simulink model "skarab_fgbe"  (R2018a)
settings: Solver=VariableStepDiscrete  StartTime=0.0  StopTime=50000  RelTol=1e-3
libraries: xbsIndex_r4 x178, xps_library x3, casper_library_misc x2
(part 3 of 3)

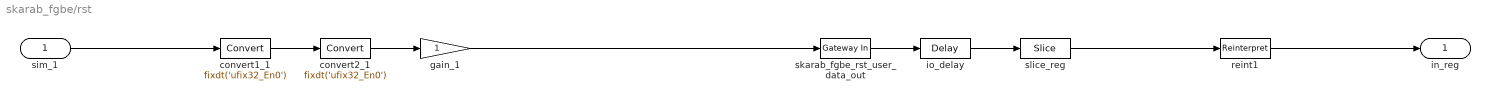
== system skarab_fgbe/rst ==
  sim_1 : Inport
  convert1_1 : DataTypeConversion  OutDataTypeStr=fixdt('ufix32_En0')  LockScale=on
  convert2_1 : DataTypeConversion  OutDataTypeStr=fixdt('ufix32_En0')  ConvertRealWorld=Stored Integer (SI)  LockScale=on
  gain_1 : Gain
  io_delay : xbsIndex_r4/Delay  rst=off  infoeditControl=Selection of Reset will increase slice count due to use of real FFs and instead of SRLs  en=off  latency=0  reg_retiming=on  dbl_ovrd=off  block_type=delay
  reint1 : xbsIndex_r4/Reinterpret  force_arith_type=on  arith_type=Unsigned  force_bin_pt=on  bin_pt=0  block_type=reinterpret
  skarab_fgbe_rst_user_data_out : xbsIndex_r4/Gateway In  gui_display_data_type=Fixed-point  arith_type=Unsigned  n_bits=32  bin_pt=0  preci_type=Single  exp_width=8  frac_width=24  rows=1  columns=1  quantization="Round  (unbiased: +/- Inf)"  overflow=Saturate  period=1  UseAsADC=off  ADCChannel='1'  interface=None  automatic_assignment=on  address_offset=hex2dec('00')  intf_name=''  intf_description=''  default_value=0  timing_constraint=None  locs_specified=off  LOCs={}  io_standard={}  inherit_from_input=off  hdl_port=on  dbl_ovrd=off  block_type=gatewayin
  slice_reg : xbsIndex_r4/Slice  nbits=32  boolean_output=off  mode=Lower Bit Location + Width  bit1=0  base1=MSB of Input  bit0=0  base0=LSB of Input  dbl_ovrd=off  block_type=slice
  in_reg : Outport
  wires:
  skarab_fgbe_rst_user_data_out/1 -> io_delay/1
  sim_1/1 -> convert1_1/1
  convert1_1/1 -> convert2_1/1
  convert2_1/1 -> gain_1/1
  gain_1/1 -> skarab_fgbe_rst_user_data_out/1
  io_delay/1 -> slice_reg/1
  slice_reg/1 -> reint1/1
  reint1/1 -> in_reg/1

== system skarab_fgbe/rx ==
  out_reg : Inport
  assert_reg : xbsIndex_r4/Assert  assert_type=on  type_source=Explicitly  gui_display_data_type=Fixed-point  arith_type=Unsigned  n_bits=32  bin_pt=0  preci_type=Single  exp_width=8  frac_width=24  assert_rate=off  rate_source=Explicitly  period=1  output_port=on  block_type=assert
  cast_gw : xbsIndex_r4/Convert  gui_display_data_type=Fixed-point  arith_type=Unsigned  n_bits=32  bin_pt=0  float_type=Single  exp_bits=8  fraction_bits=24  quantization=Truncate  overflow=Wrap  en=off  latency=1  pipeline=off  dbl_ovrd=off  block_type=convert
  io_delay : xbsIndex_r4/Delay  rst=off  infoeditControl=Selection of Reset will increase slice count due to use of real FFs and instead of SRLs  en=off  latency=0  reg_retiming=on  dbl_ovrd=off  block_type=delay
  reint1 : xbsIndex_r4/Reinterpret  force_arith_type=on  arith_type=Unsigned  force_bin_pt=on  bin_pt=0  block_type=reinterpret
  skarab_fgbe_rx_user_data_in : xbsIndex_r4/Gateway Out  inherit_from_input=off  hdl_port=on  rows=1  columns=1  UseAsDAC=off  DACChannel='1'  interface=None  automatic_assignment=on  address_offset=hex2dec('00')  intf_name=''  intf_description=''  timing_constraint=None  locs_specified=off  LOCs={}  io_standard={}  block_type=gatewayout
  sim_out : Outport
  wires:
  io_delay/1 -> cast_gw/1
  cast_gw/1 -> skarab_fgbe_rx_user_data_in/1
  skarab_fgbe_rx_user_data_in/1 -> sim_out/1
  out_reg/1 -> assert_reg/1
  assert_reg/1 -> reint1/1
  reint1/1 -> io_delay/1

== system skarab_fgbe/rx_bad_frame ==
  out_reg : Inport
  assert_reg : xbsIndex_r4/Assert  assert_type=on  type_source=Explicitly  gui_display_data_type=Fixed-point  arith_type=Unsigned  n_bits=32  bin_pt=0  preci_type=Single  exp_width=8  frac_width=24  assert_rate=off  rate_source=Explicitly  period=1  output_port=on  block_type=assert
  cast_gw : xbsIndex_r4/Convert  gui_display_data_type=Fixed-point  arith_type=Unsigned  n_bits=32  bin_pt=0  float_type=Single  exp_bits=8  fraction_bits=24  quantization=Truncate  overflow=Wrap  en=off  latency=1  pipeline=off  dbl_ovrd=off  block_type=convert
  io_delay : xbsIndex_r4/Delay  rst=off  infoeditControl=Selection of Reset will increase slice count due to use of real FFs and instead of SRLs  en=off  latency=0  reg_retiming=on  dbl_ovrd=off  block_type=delay
  reint1 : xbsIndex_r4/Reinterpret  force_arith_type=on  arith_type=Unsigned  force_bin_pt=on  bin_pt=0  block_type=reinterpret
  skarab_fgbe_rx_bad_frame_user_data_in : xbsIndex_r4/Gateway Out  inherit_from_input=off  hdl_port=on  rows=1  columns=1  UseAsDAC=off  DACChannel='1'  interface=None  automatic_assignment=on  address_offset=hex2dec('00')  intf_name=''  intf_description=''  timing_constraint=None  locs_specified=off  LOCs={}  io_standard={}  block_type=gatewayout
  sim_out : Outport
  wires:
  io_delay/1 -> cast_gw/1
  cast_gw/1 -> skarab_fgbe_rx_bad_frame_user_data_in/1
  skarab_fgbe_rx_bad_frame_user_data_in/1 -> sim_out/1
  out_reg/1 -> assert_reg/1
  assert_reg/1 -> reint1/1
  reint1/1 -> io_delay/1

== system skarab_fgbe/rx_data ==
  out_reg : Inport
  assert_reg : xbsIndex_r4/Assert  assert_type=on  type_source=Explicitly  gui_display_data_type=Fixed-point  arith_type=Unsigned  n_bits=32  bin_pt=0  preci_type=Single  exp_width=8  frac_width=24  assert_rate=off  rate_source=Explicitly  period=1  output_port=on  block_type=assert
  cast_gw : xbsIndex_r4/Convert  gui_display_data_type=Fixed-point  arith_type=Unsigned  n_bits=32  bin_pt=0  float_type=Single  exp_bits=8  fraction_bits=24  quantization=Truncate  overflow=Wrap  en=off  latency=1  pipeline=off  dbl_ovrd=off  block_type=convert
  io_delay : xbsIndex_r4/Delay  rst=off  infoeditControl=Selection of Reset will increase slice count due to use of real FFs and instead of SRLs  en=off  latency=0  reg_retiming=on  dbl_ovrd=off  block_type=delay
  reint1 : xbsIndex_r4/Reinterpret  force_arith_type=on  arith_type=Unsigned  force_bin_pt=on  bin_pt=0  block_type=reinterpret
  skarab_fgbe_rx_data_user_data_in : xbsIndex_r4/Gateway Out  inherit_from_input=off  hdl_port=on  rows=1  columns=1  UseAsDAC=off  DACChannel='1'  interface=None  automatic_assignment=on  address_offset=hex2dec('00')  intf_name=''  intf_description=''  timing_constraint=None  locs_specified=off  LOCs={}  io_standard={}  block_type=gatewayout
  sim_out : Outport
  wires:
  io_delay/1 -> cast_gw/1
  cast_gw/1 -> skarab_fgbe_rx_data_user_data_in/1
  skarab_fgbe_rx_data_user_data_in/1 -> sim_out/1
  out_reg/1 -> assert_reg/1
  assert_reg/1 -> reint1/1
  reint1/1 -> io_delay/1

== system skarab_fgbe/rx_dest_ip ==
  out_reg : Inport
  assert_reg : xbsIndex_r4/Assert  assert_type=on  type_source=Explicitly  gui_display_data_type=Fixed-point  arith_type=Unsigned  n_bits=32  bin_pt=0  preci_type=Single  exp_width=8  frac_width=24  assert_rate=off  rate_source=Explicitly  period=1  output_port=on  block_type=assert
  cast_gw : xbsIndex_r4/Convert  gui_display_data_type=Fixed-point  arith_type=Unsigned  n_bits=32  bin_pt=0  float_type=Single  exp_bits=8  fraction_bits=24  quantization=Truncate  overflow=Wrap  en=off  latency=1  pipeline=off  dbl_ovrd=off  block_type=convert
  io_delay : xbsIndex_r4/Delay  rst=off  infoeditControl=Selection of Reset will increase slice count due to use of real FFs and instead of SRLs  en=off  latency=0  reg_retiming=on  dbl_ovrd=off  block_type=delay
  reint1 : xbsIndex_r4/Reinterpret  force_arith_type=on  arith_type=Unsigned  force_bin_pt=on  bin_pt=0  block_type=reinterpret
  skarab_fgbe_rx_dest_ip_user_data_in : xbsIndex_r4/Gateway Out  inherit_from_input=off  hdl_port=on  rows=1  columns=1  UseAsDAC=off  DACChannel='1'  interface=None  automatic_assignment=on  address_offset=hex2dec('00')  intf_name=''  intf_description=''  timing_constraint=None  locs_specified=off  LOCs={}  io_standard={}  block_type=gatewayout
  sim_out : Outport
  wires:
  io_delay/1 -> cast_gw/1
  cast_gw/1 -> skarab_fgbe_rx_dest_ip_user_data_in/1
  skarab_fgbe_rx_dest_ip_user_data_in/1 -> sim_out/1
  out_reg/1 -> assert_reg/1
  assert_reg/1 -> reint1/1
  reint1/1 -> io_delay/1

== system skarab_fgbe/rx_dest_port ==
  out_reg : Inport
  assert_reg : xbsIndex_r4/Assert  assert_type=on  type_source=Explicitly  gui_display_data_type=Fixed-point  arith_type=Unsigned  n_bits=32  bin_pt=0  preci_type=Single  exp_width=8  frac_width=24  assert_rate=off  rate_source=Explicitly  period=1  output_port=on  block_type=assert
  cast_gw : xbsIndex_r4/Convert  gui_display_data_type=Fixed-point  arith_type=Unsigned  n_bits=32  bin_pt=0  float_type=Single  exp_bits=8  fraction_bits=24  quantization=Truncate  overflow=Wrap  en=off  latency=1  pipeline=off  dbl_ovrd=off  block_type=convert
  io_delay : xbsIndex_r4/Delay  rst=off  infoeditControl=Selection of Reset will increase slice count due to use of real FFs and instead of SRLs  en=off  latency=0  reg_retiming=on  dbl_ovrd=off  block_type=delay
  reint1 : xbsIndex_r4/Reinterpret  force_arith_type=on  arith_type=Unsigned  force_bin_pt=on  bin_pt=0  block_type=reinterpret
  skarab_fgbe_rx_dest_port_user_data_in : xbsIndex_r4/Gateway Out  inherit_from_input=off  hdl_port=on  rows=1  columns=1  UseAsDAC=off  DACChannel='1'  interface=None  automatic_assignment=on  address_offset=hex2dec('00')  intf_name=''  intf_description=''  timing_constraint=None  locs_specified=off  LOCs={}  io_standard={}  block_type=gatewayout
  sim_out : Outport
  wires:
  io_delay/1 -> cast_gw/1
  cast_gw/1 -> skarab_fgbe_rx_dest_port_user_data_in/1
  skarab_fgbe_rx_dest_port_user_data_in/1 -> sim_out/1
  out_reg/1 -> assert_reg/1
  assert_reg/1 -> reint1/1
  reint1/1 -> io_delay/1

== system skarab_fgbe/rx_end_of_frame ==
  out_reg : Inport
  assert_reg : xbsIndex_r4/Assert  assert_type=on  type_source=Explicitly  gui_display_data_type=Fixed-point  arith_type=Unsigned  n_bits=32  bin_pt=0  preci_type=Single  exp_width=8  frac_width=24  assert_rate=off  rate_source=Explicitly  period=1  output_port=on  block_type=assert
  cast_gw : xbsIndex_r4/Convert  gui_display_data_type=Fixed-point  arith_type=Unsigned  n_bits=32  bin_pt=0  float_type=Single  exp_bits=8  fraction_bits=24  quantization=Truncate  overflow=Wrap  en=off  latency=1  pipeline=off  dbl_ovrd=off  block_type=convert
  io_delay : xbsIndex_r4/Delay  rst=off  infoeditControl=Selection of Reset will increase slice count due to use of real FFs and instead of SRLs  en=off  latency=0  reg_retiming=on  dbl_ovrd=off  block_type=delay
  reint1 : xbsIndex_r4/Reinterpret  force_arith_type=on  arith_type=Unsigned  force_bin_pt=on  bin_pt=0  block_type=reinterpret
  skarab_fgbe_rx_end_of_frame_user_data_in : xbsIndex_r4/Gateway Out  inherit_from_input=off  hdl_port=on  rows=1  columns=1  UseAsDAC=off  DACChannel='1'  interface=None  automatic_assignment=on  address_offset=hex2dec('00')  intf_name=''  intf_description=''  timing_constraint=None  locs_specified=off  LOCs={}  io_standard={}  block_type=gatewayout
  sim_out : Outport
  wires:
  io_delay/1 -> cast_gw/1
  cast_gw/1 -> skarab_fgbe_rx_end_of_frame_user_data_in/1
  skarab_fgbe_rx_end_of_frame_user_data_in/1 -> sim_out/1
  out_reg/1 -> assert_reg/1
  assert_reg/1 -> reint1/1
  reint1/1 -> io_delay/1

== system skarab_fgbe/rx_valid ==
  out_reg : Inport
  assert_reg : xbsIndex_r4/Assert  assert_type=on  type_source=Explicitly  gui_display_data_type=Fixed-point  arith_type=Unsigned  n_bits=32  bin_pt=0  preci_type=Single  exp_width=8  frac_width=24  assert_rate=off  rate_source=Explicitly  period=1  output_port=on  block_type=assert
  cast_gw : xbsIndex_r4/Convert  gui_display_data_type=Fixed-point  arith_type=Unsigned  n_bits=32  bin_pt=0  float_type=Single  exp_bits=8  fraction_bits=24  quantization=Truncate  overflow=Wrap  en=off  latency=1  pipeline=off  dbl_ovrd=off  block_type=convert
  io_delay : xbsIndex_r4/Delay  rst=off  infoeditControl=Selection of Reset will increase slice count due to use of real FFs and instead of SRLs  en=off  latency=0  reg_retiming=on  dbl_ovrd=off  block_type=delay
  reint1 : xbsIndex_r4/Reinterpret  force_arith_type=on  arith_type=Unsigned  force_bin_pt=on  bin_pt=0  block_type=reinterpret
  skarab_fgbe_rx_valid_user_data_in : xbsIndex_r4/Gateway Out  inherit_from_input=off  hdl_port=on  rows=1  columns=1  UseAsDAC=off  DACChannel='1'  interface=None  automatic_assignment=on  address_offset=hex2dec('00')  intf_name=''  intf_description=''  timing_constraint=None  locs_specified=off  LOCs={}  io_standard={}  block_type=gatewayout
  sim_out : Outport
  wires:
  io_delay/1 -> cast_gw/1
  cast_gw/1 -> skarab_fgbe_rx_valid_user_data_in/1
  skarab_fgbe_rx_valid_user_data_in/1 -> sim_out/1
  out_reg/1 -> assert_reg/1
  assert_reg/1 -> reint1/1
  reint1/1 -> io_delay/1

== system skarab_fgbe/tx ==
  out_reg : Inport
  assert_reg : xbsIndex_r4/Assert  assert_type=on  type_source=Explicitly  gui_display_data_type=Fixed-point  arith_type=Unsigned  n_bits=32  bin_pt=0  preci_type=Single  exp_width=8  frac_width=24  assert_rate=off  rate_source=Explicitly  period=1  output_port=on  block_type=assert
  cast_gw : xbsIndex_r4/Convert  gui_display_data_type=Fixed-point  arith_type=Unsigned  n_bits=32  bin_pt=0  float_type=Single  exp_bits=8  fraction_bits=24  quantization=Truncate  overflow=Wrap  en=off  latency=1  pipeline=off  dbl_ovrd=off  block_type=convert
  io_delay : xbsIndex_r4/Delay  rst=off  infoeditControl=Selection of Reset will increase slice count due to use of real FFs and instead of SRLs  en=off  latency=0  reg_retiming=on  dbl_ovrd=off  block_type=delay
  reint1 : xbsIndex_r4/Reinterpret  force_arith_type=on  arith_type=Unsigned  force_bin_pt=on  bin_pt=0  block_type=reinterpret
  skarab_fgbe_tx_user_data_in : xbsIndex_r4/Gateway Out  inherit_from_input=off  hdl_port=on  rows=1  columns=1  UseAsDAC=off  DACChannel='1'  interface=None  automatic_assignment=on  address_offset=hex2dec('00')  intf_name=''  intf_description=''  timing_constraint=None  locs_specified=off  LOCs={}  io_standard={}  block_type=gatewayout
  sim_out : Outport
  wires:
  io_delay/1 -> cast_gw/1
  cast_gw/1 -> skarab_fgbe_tx_user_data_in/1
  skarab_fgbe_tx_user_data_in/1 -> sim_out/1
  out_reg/1 -> assert_reg/1
  assert_reg/1 -> reint1/1
  reint1/1 -> io_delay/1

== system skarab_fgbe/tx_cnt ==
  out_reg : Inport
  assert_reg : xbsIndex_r4/Assert  assert_type=on  type_source=Explicitly  gui_display_data_type=Fixed-point  arith_type=Unsigned  n_bits=32  bin_pt=0  preci_type=Single  exp_width=8  frac_width=24  assert_rate=off  rate_source=Explicitly  period=1  output_port=on  block_type=assert
  cast_gw : xbsIndex_r4/Convert  gui_display_data_type=Fixed-point  arith_type=Unsigned  n_bits=32  bin_pt=0  float_type=Single  exp_bits=8  fraction_bits=24  quantization=Truncate  overflow=Wrap  en=off  latency=1  pipeline=off  dbl_ovrd=off  block_type=convert
  io_delay : xbsIndex_r4/Delay  rst=off  infoeditControl=Selection of Reset will increase slice count due to use of real FFs and instead of SRLs  en=off  latency=0  reg_retiming=on  dbl_ovrd=off  block_type=delay
  reint1 : xbsIndex_r4/Reinterpret  force_arith_type=on  arith_type=Unsigned  force_bin_pt=on  bin_pt=0  block_type=reinterpret
  skarab_fgbe_tx_cnt_user_data_in : xbsIndex_r4/Gateway Out  inherit_from_input=off  hdl_port=on  rows=1  columns=1  UseAsDAC=off  DACChannel='1'  interface=None  automatic_assignment=on  address_offset=hex2dec('00')  intf_name=''  intf_description=''  timing_constraint=None  locs_specified=off  LOCs={}  io_standard={}  block_type=gatewayout
  sim_out : Outport
  wires:
  io_delay/1 -> cast_gw/1
  cast_gw/1 -> skarab_fgbe_tx_cnt_user_data_in/1
  skarab_fgbe_tx_cnt_user_data_in/1 -> sim_out/1
  out_reg/1 -> assert_reg/1
  assert_reg/1 -> reint1/1
  reint1/1 -> io_delay/1

== system skarab_fgbe/tx_full ==
  out_reg : Inport
  assert_reg : xbsIndex_r4/Assert  assert_type=on  type_source=Explicitly  gui_display_data_type=Fixed-point  arith_type=Unsigned  n_bits=32  bin_pt=0  preci_type=Single  exp_width=8  frac_width=24  assert_rate=off  rate_source=Explicitly  period=1  output_port=on  block_type=assert
  cast_gw : xbsIndex_r4/Convert  gui_display_data_type=Fixed-point  arith_type=Unsigned  n_bits=32  bin_pt=0  float_type=Single  exp_bits=8  fraction_bits=24  quantization=Truncate  overflow=Wrap  en=off  latency=1  pipeline=off  dbl_ovrd=off  block_type=convert
  io_delay : xbsIndex_r4/Delay  rst=off  infoeditControl=Selection of Reset will increase slice count due to use of real FFs and instead of SRLs  en=off  latency=0  reg_retiming=on  dbl_ovrd=off  block_type=delay
  reint1 : xbsIndex_r4/Reinterpret  force_arith_type=on  arith_type=Unsigned  force_bin_pt=on  bin_pt=0  block_type=reinterpret
  skarab_fgbe_tx_full_user_data_in : xbsIndex_r4/Gateway Out  inherit_from_input=off  hdl_port=on  rows=1  columns=1  UseAsDAC=off  DACChannel='1'  interface=None  automatic_assignment=on  address_offset=hex2dec('00')  intf_name=''  intf_description=''  timing_constraint=None  locs_specified=off  LOCs={}  io_standard={}  block_type=gatewayout
  sim_out : Outport
  wires:
  io_delay/1 -> cast_gw/1
  cast_gw/1 -> skarab_fgbe_tx_full_user_data_in/1
  skarab_fgbe_tx_full_user_data_in/1 -> sim_out/1
  out_reg/1 -> assert_reg/1
  assert_reg/1 -> reint1/1
  reint1/1 -> io_delay/1

== system skarab_fgbe/tx_overflow ==
  out_reg : Inport
  assert_reg : xbsIndex_r4/Assert  assert_type=on  type_source=Explicitly  gui_display_data_type=Fixed-point  arith_type=Unsigned  n_bits=32  bin_pt=0  preci_type=Single  exp_width=8  frac_width=24  assert_rate=off  rate_source=Explicitly  period=1  output_port=on  block_type=assert
  cast_gw : xbsIndex_r4/Convert  gui_display_data_type=Fixed-point  arith_type=Unsigned  n_bits=32  bin_pt=0  float_type=Single  exp_bits=8  fraction_bits=24  quantization=Truncate  overflow=Wrap  en=off  latency=1  pipeline=off  dbl_ovrd=off  block_type=convert
  io_delay : xbsIndex_r4/Delay  rst=off  infoeditControl=Selection of Reset will increase slice count due to use of real FFs and instead of SRLs  en=off  latency=0  reg_retiming=on  dbl_ovrd=off  block_type=delay
  reint1 : xbsIndex_r4/Reinterpret  force_arith_type=on  arith_type=Unsigned  force_bin_pt=on  bin_pt=0  block_type=reinterpret
  skarab_fgbe_tx_overflow_user_data_in : xbsIndex_r4/Gateway Out  inherit_from_input=off  hdl_port=on  rows=1  columns=1  UseAsDAC=off  DACChannel='1'  interface=None  automatic_assignment=on  address_offset=hex2dec('00')  intf_name=''  intf_description=''  timing_constraint=None  locs_specified=off  LOCs={}  io_standard={}  block_type=gatewayout
  sim_out : Outport
  wires:
  io_delay/1 -> cast_gw/1
  cast_gw/1 -> skarab_fgbe_tx_overflow_user_data_in/1
  skarab_fgbe_tx_overflow_user_data_in/1 -> sim_out/1
  out_reg/1 -> assert_reg/1
  assert_reg/1 -> reint1/1
  reint1/1 -> io_delay/1

== system skarab_fgbe/forty_gbe/convert_tx_valid ==
  in : Inport
  bussify : Subsystem  AncestorBlock=casper_library_flow_control/bus_create  mask(bus_create){inputNum=4}
      mask prompts: inputNum "Number of inputs:"
      mask init:
      | bus_create_init(gcb,...
      |     'inputNum', inputNum);
  out : Outport
  wires:
  in/1 -> bussify/1(in1), bussify/2(in2), bussify/3(in3), bussify/4(in4)
  bussify/1(bus_out) -> out/1

== system skarab_fgbe/forty_gbe/pipeline_led_rx ==
  d : Inport
  q : Outport
  wires:
  d/1 -> q/1

== system skarab_fgbe/forty_gbe/pipeline_led_tx ==
  d : Inport
  q : Outport
  wires:
  d/1 -> q/1

== system skarab_fgbe/forty_gbe/pipeline_led_up ==
  d : Inport
  q : Outport
  wires:
  d/1 -> q/1

== system skarab_fgbe/forty_gbe/pipeline_rx_bad_frame ==
  d : Inport
  q : Outport
  wires:
  d/1 -> q/1

== system skarab_fgbe/forty_gbe/pipeline_rx_data ==
  d : Inport
  q : Outport
  wires:
  d/1 -> q/1

== system skarab_fgbe/forty_gbe/pipeline_rx_dest_ip ==
  d : Inport
  q : Outport
  wires:
  d/1 -> q/1

== system skarab_fgbe/forty_gbe/pipeline_rx_dest_port ==
  d : Inport
  q : Outport
  wires:
  d/1 -> q/1

== system skarab_fgbe/forty_gbe/pipeline_rx_end_of_frame ==
  d : Inport
  q : Outport
  wires:
  d/1 -> q/1

== system skarab_fgbe/forty_gbe/pipeline_rx_overrun ==
  d : Inport
  q : Outport
  wires:
  d/1 -> q/1

== system skarab_fgbe/forty_gbe/pipeline_rx_source_ip ==
  d : Inport
  q : Outport
  wires:
  d/1 -> q/1

== system skarab_fgbe/forty_gbe/pipeline_rx_source_port ==
  d : Inport
  q : Outport
  wires:
  d/1 -> q/1

== system skarab_fgbe/forty_gbe/pipeline_rx_valid ==
  d : Inport
  q : Outport
  wires:
  d/1 -> q/1

== system skarab_fgbe/forty_gbe/pipeline_tx_afull ==
  d : Inport
  q : Outport
  wires:
  d/1 -> q/1

== system skarab_fgbe/forty_gbe/pipeline_tx_overflow ==
  d : Inport
  q : Outport
  wires:
  d/1 -> q/1

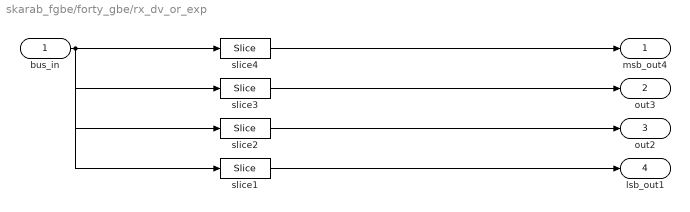
== system skarab_fgbe/forty_gbe/rx_dv_or_exp ==
  bus_in : Inport
  slice1 : xbsIndex_r4/Slice  nbits=1  boolean_output=on  mode=Upper Bit Location + Width  bit1=-3  base1=MSB of Input  bit0=0  base0=LSB of Input  dbl_ovrd=off  block_type=slice
  slice2 : xbsIndex_r4/Slice  nbits=1  boolean_output=on  mode=Upper Bit Location + Width  bit1=-2  base1=MSB of Input  bit0=0  base0=LSB of Input  dbl_ovrd=off  block_type=slice
  slice3 : xbsIndex_r4/Slice  nbits=1  boolean_output=on  mode=Upper Bit Location + Width  bit1=-1  base1=MSB of Input  bit0=0  base0=LSB of Input  dbl_ovrd=off  block_type=slice
  slice4 : xbsIndex_r4/Slice  nbits=1  boolean_output=on  mode=Upper Bit Location + Width  bit1=0  base1=MSB of Input  bit0=0  base0=LSB of Input  dbl_ovrd=off  block_type=slice
  msb_out4 : Outport
  out3 : Outport  Port=2
  out2 : Outport  Port=3
  lsb_out1 : Outport  Port=4
  wires:
  bus_in/1 -> slice4/1, slice3/1, slice2/1, slice1/1
  slice4/1 -> msb_out4/1
  slice3/1 -> out3/1
  slice2/1 -> out2/1
  slice1/1 -> lsb_out1/1

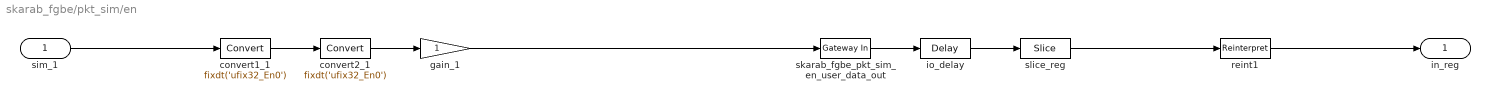
== system skarab_fgbe/pkt_sim/en ==
  sim_1 : Inport
  convert1_1 : DataTypeConversion  OutDataTypeStr=fixdt('ufix32_En0')  LockScale=on
  convert2_1 : DataTypeConversion  OutDataTypeStr=fixdt('ufix32_En0')  ConvertRealWorld=Stored Integer (SI)  LockScale=on
  gain_1 : Gain
  io_delay : xbsIndex_r4/Delay  rst=off  infoeditControl=Selection of Reset will increase slice count due to use of real FFs and instead of SRLs  en=off  latency=0  reg_retiming=on  dbl_ovrd=off  block_type=delay
  reint1 : xbsIndex_r4/Reinterpret  force_arith_type=on  arith_type=Unsigned  force_bin_pt=on  bin_pt=0  block_type=reinterpret
  skarab_fgbe_pkt_sim_en_user_data_out : xbsIndex_r4/Gateway In  gui_display_data_type=Fixed-point  arith_type=Unsigned  n_bits=32  bin_pt=0  preci_type=Single  exp_width=8  frac_width=24  rows=1  columns=1  quantization="Round  (unbiased: +/- Inf)"  overflow=Saturate  period=1  UseAsADC=off  ADCChannel='1'  interface=None  automatic_assignment=on  address_offset=hex2dec('00')  intf_name=''  intf_description=''  default_value=0  timing_constraint=None  locs_specified=off  LOCs={}  io_standard={}  inherit_from_input=off  hdl_port=on  dbl_ovrd=off  block_type=gatewayin
  slice_reg : xbsIndex_r4/Slice  nbits=32  boolean_output=off  mode=Lower Bit Location + Width  bit1=0  base1=MSB of Input  bit0=0  base0=LSB of Input  dbl_ovrd=off  block_type=slice
  in_reg : Outport
  wires:
  skarab_fgbe_pkt_sim_en_user_data_out/1 -> io_delay/1
  sim_1/1 -> convert1_1/1
  convert1_1/1 -> convert2_1/1
  convert2_1/1 -> gain_1/1
  gain_1/1 -> skarab_fgbe_pkt_sim_en_user_data_out/1
  io_delay/1 -> slice_reg/1
  slice_reg/1 -> reint1/1
  reint1/1 -> in_reg/1

== system skarab_fgbe/pkt_sim/negedge ==
  in : Inport
  Delay : xbsIndex_r4/Delay  rst=off  infoeditControl=Selection of Reset will increase slice count due to use of real FFs and instead of SRLs  en=off  latency=1  reg_retiming=off  dbl_ovrd=off  block_type=delay
      settings: xl_area=[0, 0, 0, 0, 0, 0, 0]
  Inverter : xbsIndex_r4/Inverter  en=off  latency=0  dbl_ovrd=off  block_type=inv
      settings: xl_area=[0, 0, 0, 0, 0, 0, 0]
  edge_op : xbsIndex_r4/Logical  logical_function=AND  inputs=2  en=off  latency=0  precision=Full  arith_type=Unsigned  n_bits=8  bin_pt=2  align_bp=on  dbl_ovrd=off  block_type=logical
      settings: xl_area=[0, 0, 0, 0, 0, 0, 0]
  out : Outport
  wires:
  Inverter/1 -> edge_op/1
  edge_op/1 -> out/1
  in/1 -> Inverter/1, Delay/1
  Delay/1 -> edge_op/2

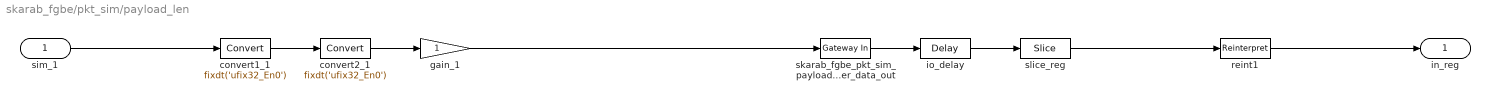
== system skarab_fgbe/pkt_sim/payload_len ==
  sim_1 : Inport
  convert1_1 : DataTypeConversion  OutDataTypeStr=fixdt('ufix32_En0')  LockScale=on
  convert2_1 : DataTypeConversion  OutDataTypeStr=fixdt('ufix32_En0')  ConvertRealWorld=Stored Integer (SI)  LockScale=on
  gain_1 : Gain
  io_delay : xbsIndex_r4/Delay  rst=off  infoeditControl=Selection of Reset will increase slice count due to use of real FFs and instead of SRLs  en=off  latency=0  reg_retiming=on  dbl_ovrd=off  block_type=delay
  reint1 : xbsIndex_r4/Reinterpret  force_arith_type=on  arith_type=Unsigned  force_bin_pt=on  bin_pt=0  block_type=reinterpret
  skarab_fgbe_pkt_sim_payload_len_user_data_out : xbsIndex_r4/Gateway In  gui_display_data_type=Fixed-point  arith_type=Unsigned  n_bits=32  bin_pt=0  preci_type=Single  exp_width=8  frac_width=24  rows=1  columns=1  quantization="Round  (unbiased: +/- Inf)"  overflow=Saturate  period=1  UseAsADC=off  ADCChannel='1'  interface=None  automatic_assignment=on  address_offset=hex2dec('00')  intf_name=''  intf_description=''  default_value=0  timing_constraint=None  locs_specified=off  LOCs={}  io_standard={}  inherit_from_input=off  hdl_port=on  dbl_ovrd=off  block_type=gatewayin
  slice_reg : xbsIndex_r4/Slice  nbits=32  boolean_output=off  mode=Lower Bit Location + Width  bit1=0  base1=MSB of Input  bit0=0  base0=LSB of Input  dbl_ovrd=off  block_type=slice
  in_reg : Outport
  wires:
  skarab_fgbe_pkt_sim_payload_len_user_data_out/1 -> io_delay/1
  sim_1/1 -> convert1_1/1
  convert1_1/1 -> convert2_1/1
  convert2_1/1 -> gain_1/1
  gain_1/1 -> skarab_fgbe_pkt_sim_payload_len_user_data_out/1
  io_delay/1 -> slice_reg/1
  slice_reg/1 -> reint1/1
  reint1/1 -> in_reg/1

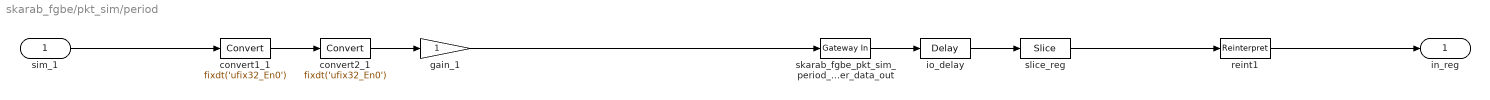
== system skarab_fgbe/pkt_sim/period ==
  sim_1 : Inport
  convert1_1 : DataTypeConversion  OutDataTypeStr=fixdt('ufix32_En0')  LockScale=on
  convert2_1 : DataTypeConversion  OutDataTypeStr=fixdt('ufix32_En0')  ConvertRealWorld=Stored Integer (SI)  LockScale=on
  gain_1 : Gain
  io_delay : xbsIndex_r4/Delay  rst=off  infoeditControl=Selection of Reset will increase slice count due to use of real FFs and instead of SRLs  en=off  latency=0  reg_retiming=on  dbl_ovrd=off  block_type=delay
  reint1 : xbsIndex_r4/Reinterpret  force_arith_type=on  arith_type=Unsigned  force_bin_pt=on  bin_pt=0  block_type=reinterpret
  skarab_fgbe_pkt_sim_period_user_data_out : xbsIndex_r4/Gateway In  gui_display_data_type=Fixed-point  arith_type=Unsigned  n_bits=32  bin_pt=0  preci_type=Single  exp_width=8  frac_width=24  rows=1  columns=1  quantization="Round  (unbiased: +/- Inf)"  overflow=Saturate  period=1  UseAsADC=off  ADCChannel='1'  interface=None  automatic_assignment=on  address_offset=hex2dec('00')  intf_name=''  intf_description=''  default_value=0  timing_constraint=None  locs_specified=off  LOCs={}  io_standard={}  inherit_from_input=off  hdl_port=on  dbl_ovrd=off  block_type=gatewayin
  slice_reg : xbsIndex_r4/Slice  nbits=32  boolean_output=off  mode=Lower Bit Location + Width  bit1=0  base1=MSB of Input  bit0=0  base0=LSB of Input  dbl_ovrd=off  block_type=slice
  in_reg : Outport
  wires:
  skarab_fgbe_pkt_sim_period_user_data_out/1 -> io_delay/1
  sim_1/1 -> convert1_1/1
  convert1_1/1 -> convert2_1/1
  convert2_1/1 -> gain_1/1
  gain_1/1 -> skarab_fgbe_pkt_sim_period_user_data_out/1
  io_delay/1 -> slice_reg/1
  slice_reg/1 -> reint1/1
  reint1/1 -> in_reg/1

== system skarab_fgbe/pkt_sim/posedge ==
  in : Inport
  Delay : xbsIndex_r4/Delay  rst=off  infoeditControl=Selection of Reset will increase slice count due to use of real FFs and instead of SRLs  en=off  latency=1  reg_retiming=off  dbl_ovrd=off  block_type=delay
      settings: xl_area=[0, 0, 0, 0, 0, 0, 0]
  Inverter : xbsIndex_r4/Inverter  en=off  latency=0  dbl_ovrd=off  block_type=inv
      settings: xl_area=[0, 0, 0, 0, 0, 0, 0]
  edge_op : xbsIndex_r4/Logical  logical_function=NOR  inputs=2  en=off  latency=0  precision=Full  arith_type=Unsigned  n_bits=8  bin_pt=2  align_bp=on  dbl_ovrd=off  block_type=logical
      settings: xl_area=[0, 0, 0, 0, 0, 0, 0]
  out : Outport
  wires:
  Inverter/1 -> edge_op/1
  edge_op/1 -> out/1
  in/1 -> Inverter/1, Delay/1
  Delay/1 -> edge_op/2

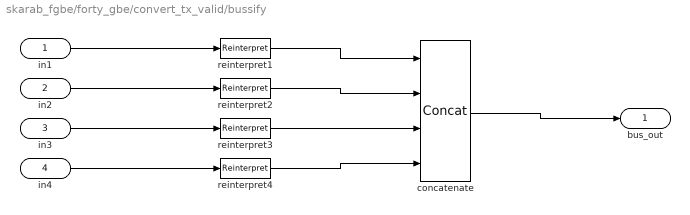
== system skarab_fgbe/forty_gbe/convert_tx_valid/bussify ==
  in1 : Inport
  in2 : Inport  Port=2
  in3 : Inport  Port=3
  in4 : Inport  Port=4
  concatenate : xbsIndex_r4/Concat  num_inputs=4  dbl_ovrd=off  block_type=concat
  reinterpret{1..4} (4 alike) : xbsIndex_r4/Reinterpret  force_arith_type=on  arith_type=Unsigned  force_bin_pt=on  bin_pt=0  block_type=reinterpret
      reinterpret1 settings: infoedit="Changes signal type without altering the binary representation.   You can changed the signal between signed and unsigned, and relocate the binary point.<br><br>Hardware notes: In hardware this block costs nothing.<br><br>Example:  Suppose the input is 6 bits wide, signed, with 2 fractional bits, and the output is forced to unsigned with 0 fractional bits.  Then an input of -2.0 (1110.00 in binary 2's complement) becomes an output of 56 (111000 in binary)."
      reinterpret2 settings: infoedit="Changes signal type without altering the binary representation.   You can changed the signal between signed and unsigned, and relocate the binary point.<br><br>Hardware notes: In hardware this block costs nothing.<br><br>Example:  Suppose the input is 6 bits wide, signed, with 2 fractional bits, and the output is forced to unsigned with 0 fractional bits.  Then an input of -2.0 (1110.00 in binary 2's complement) becomes an output of 56 (111000 in binary)."
  bus_out : Outport
  wires:
  concatenate/1 -> bus_out/1
  in1/1 -> reinterpret1/1
  reinterpret1/1 -> concatenate/1
  in2/1 -> reinterpret2/1
  reinterpret2/1 -> concatenate/2
  in3/1 -> reinterpret3/1
  reinterpret3/1 -> concatenate/3
  in4/1 -> reinterpret4/1
  reinterpret4/1 -> concatenate/4
